simulink model "dsPIC_32MX460F512L_Explorer16_HyperSampling"  (Simulink 6.4)
settings: Solver=FixedStepDiscrete  StartTime=0.0  StopTime=10.0  FixedStep=.001  RelTol=1e-3
undefined symbols (not defined in the file or in its folder): OCmax
libraries: dsPICdrivers x7, simulink x2
settings Model: Creator=Lubin  LastModifiedBy=Administrateur
settings OptimizationCC: InlineParams=on  InlineInvariantSignals=on  EnforceIntegerDowncast=off  StateBitsets=on  DataBitsets=on  UseTempVars=on  ZeroExternalMemoryAtStartup=off  ZeroInternalMemoryAtStartup=off  InitFltsAndDblsToZero=off  OptimizeModelRefInitCode=on  LifeSpan=1
settings DebuggingCC: MultiTaskDSMMsg=error  MultiTaskCondExecSysMsg=error
settings HardwareCC: TargetHWDeviceType=32-bit Generic
settings RTWCC: SystemTargetFile=pic32.tlc  TemplateMakefile=pic32_gcc.tmf  PostCodeGenCommand=dsPIC_Compile()  Description=Embedded Target for Microchip dsPIC (real-time)  GenerateReport=on  ProcessScript=pic32_make_rtw_hook  IncludeHyperlinkInReport=on  LaunchReport=on
settings CodeAppCC: IgnoreCustomStorageClasses=off
settings STFCustomTargetCC: TargetFcnLib=ansi_tfl_tmw.mat  GenFloatMathFcnCalls=ANSI_C  ModelReferenceCompliant=off  IncludeMdlTerminateFcn=off  CombineOutputUpdateFcns=on  SuppressErrorStatus=on  ERTCustomFileBanners=on  SupportContinuousTime=off  SupportNonInlinedSFcns=off  SystemTargetFile=pic32.tlc
settings ERTTargetCC: TargetFcnLib=ansi_tfl_tmw.mat  GenFloatMathFcnCalls=ANSI_C  ModelReferenceCompliant=off  CompOptLevelCompliant=off  IncludeMdlTerminateFcn=off  SuppressErrorStatus=on  ModelStepFunctionPrototypeControlCompliant=off  ExtModeMexFile=noextcomm  InlinedParameterPlacement=NonHierarchical  ERTSrcFileBannerTemplate=dsPIC_code_template.cgt  ERTHdrFileBannerTemplate=dsPIC_code_template.cgt  ERTDataSrcFileTemplate=dsPIC_code_template.cgt  ERTDataHdrFileTemplate=dsPIC_code_template.cgt  ERTCustomFileTemplate=dsPIC_main.tlc
settings CustomProperty: DataType=string  Value=C:\PROGRA~1\MATLAB\R2008b\bin\win32\gmake

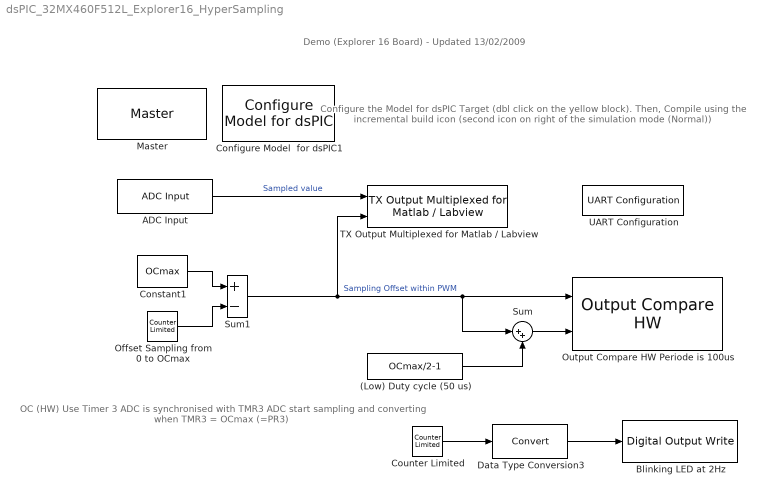
== system dsPIC_32MX460F512L_Explorer16_HyperSampling ==
  note: Demo (Explorer 16 Board) - Updated 13/02/2009
  note: Configure the Model for dsPIC Target (dbl click on the yellow block).
      | Then, Compile using the incremental build icon
      | (second icon on right of the simulation mode (Normal))
  note: OC (HW) Use Timer 3
      | ADC is synchronised with TMR3
      | ADC start sampling and converting when TMR3 = OCmax (=PR3)
  (Low) Duty cycle (50 us) : Constant  Value=OCmax/2-1  OutDataTypeMode=uint16  OutDataType=sfix(16)  OutScaling=2^0
  ADC Input : dsPICdrivers/Peripheral I//O/ADC Input  Tag=dsPIC_ADC  Priority=5  ADC_TYPE=10 bits  ADC_MODE=Continuous sampling & get last channel value  NbrSampleStep=1  VoltRefpopup="AVdd  -  AVss"  OutFormatBitspopup=0000 00dd dddd dddd : Integer  InterruptPriority=6  ANCHANNELS=5  MaxName=ANmax = 1024  Rin=5e6  ADCS=29  SAMC=31  Temperature=25  DMAChannel=0  SampleTime=.001  Status="OK  |  Tsmp=4.844e-006 |  T/Channel=6.719e-006 |  Tall=6.719e-006"  SSRC=Timer3 (OC_HW PWM)
  Blinking LED at 2Hz : dsPICdrivers/Digital I//O/Digital Output Write  Tag=dsPIC_Digital_Output  Priority=5  PORT=A  Simultaneous=off  OrderingInOutPopup=None
  Configure Model  for dsPIC1 : dsPICdrivers/Simulink Configuration/Configure Model  for dsPIC
  Constant1 : Constant  Value=OCmax  OutDataTypeMode=uint16  OutDataType=sfix(16)  OutScaling=2^0
  Counter Limited : simulink/Sources/Counter Limited  SystemSampleTime=-1  uplimit=1  tsamp=.25
  Data Type Conversion3 : DataTypeConversion  OutDataTypeMode=boolean  OutDataType=sfix(16)  OutScaling=2^0
  Master : dsPICdrivers/Master  Tag=dsPIC_MASTER  Priority=1  TimeStepType=Timer1  picType=32MX460F512L  fcy=96000000  Quartz_33f=8e6  PLLActive_33f=on  fcyDesired_33f=96e6  tmr1="[8  11999  0]"  tmr1Info="Time Step : 0.001  ;   Error : 0%  PR1=11999"  tmr2345="[0  1  0  0]"  tmr2345cfg=[-1 -1 -1 -1]  IOautoConf=on  typePort="[ 10   0   0   0   0   0   0   0   0   0   0   0   0   0   0   0   0   0   0   0   0   8   0   0   0   0   0   0   0   0   0   0   0   0   0   0   0   0   0   0   0   0   0   0   0   0   0   0  24   0   0   0   0   0   0   0   0   0   0   0   0   0   0   0   0   0   0   0   0   0   0   0   0   0   0   0   0   0   0   0   0   0   0   0   4   5   0   0   0   0   0   0   0   0   0   0   0   0   0   0   0   0   0   0   0   0   0   0   0   0   0   0 ]"  TRIS="[ 65534  65535  65535  65534  65535  65535  65535 ]"  ADPCFG=0  MasterBusyPort=None  MasterOverloadPort=None  FOSC=Quartz (XT - HS)  ClockSwitchMonitor=Both disabled  TempProtection_33f=TEMP_ON  FPBOR=<empty>  PWRT=disable  MCLR=<empty>  PowerSave=off  OverrideFcy=off  NewFcy=1e6  PR2345="[65535   9599  65535  65535]"
  Offset Sampling from 0 to OCmax : simulink/Sources/Counter Limited  SystemSampleTime=-1  uplimit=OCmax  tsamp=.001
  Output Compare HW Periode is 100us : dsPICdrivers/Peripheral I//O/Output Compare HW  Tag=dsPIC_OC_HW_out  Priority=5  OC_Mode=PWM Time Set-Reset (glitch possible)  Timer=3  CHANNEL=[1 ]  Channel_UP_Down_Periode=[16]  PeriodeInput=off  MaxChannel=0.0001  MaxName=' OCmax '  Precision=[13.2288]  Status=OK  SafeMarge=[0]  PortLetter=[68]  PortNumber=[0]  MaxValues=[9599]  NPORTS=2
  Sum : Sum  Inputs=|++  OutDataType=sfix(16)  OutScaling=2^0
  Sum1 : Sum  Inputs=+-  OutDataType=sfix(16)  OutScaling=2^0
  TX Output Multiplexed for Matlab / Labview : dsPICdrivers/Serial PORT/TX Output Multiplexed for Matlab // Labview  Tag=dsPIC_TX_Multiplexed  Priority=5  UART=2  CleverSpreadingChk=on  CleverSpreading=1  CHANNEL=[0 1]  CHANNELBLOCKED=[]  CHANNELBLOCKED_BITEWISE=0  Status=OK
  UART Configuration : dsPICdrivers/Serial PORT/UART Configuration  Tag=dsPIC_config_UART  Priority=2  UART=2  proposed_BAUD=115200  ALT_TX_RX=on  InterruptTxWhen=When Transmit Buffer is empty  TXInterruptPri=1  TxBufferSize=32  TXEN=on  InterruptRxWhen=When Receive Buffer is full (contain 4 characters)  RXInterruptPri=2  RxBufferSize=32  BAUD=115200  UxBRG=51  Info="UxBRG = 51   ||  Real Baud : 115385   ||  % error : 0.16026  ||  max 11.5385 Bytes / Step"  RealBaud=0
  wires:
  Counter Limited/1 -> Data Type Conversion3/1
  ADC Input/1 -> TX Output Multiplexed for Matlab / Labview/1  "Sampled value"
  (Low) Duty cycle (50 us)/1 -> Sum/2
  Sum/1 -> Output Compare HW Periode is 100us/2
  Sum1/1 -> Output Compare HW Periode is 100us/1, Sum/1, TX Output Multiplexed for Matlab / Labview/2  "Sampling Offset within PWM"
  Constant1/1 -> Sum1/1
  Offset Sampling from 0 to OCmax/1 -> Sum1/2
  Data Type Conversion3/1 -> Blinking LED at 2Hz/1
